simulink model "generator_loaded"  (R2021a)
settings: Solver=FixedStepAuto  StartTime=0.0  StopTime=5  FixedStep=1e-4  RelTol=1e-3
values from neighbouring files (symbols this model uses):
  f = 0.59e-4    (= 5.9e-05)    [generator_parameters.m]
  Ji = 1.15e-3    (= 0.00115)    [generator_parameters.m]
  ld = 5e-3    (= 0.005)    [generator_parameters.m]
  lq = 5e-3    (= 0.005)    [generator_parameters.m]
  p = 5    [generator_parameters.m]
  phi = 0.27    [generator_parameters.m]
  rs = 0.5    [generator_parameters.m]
libraries: spsControlledCurrentSourceLib x3, spsSeriesRLCBranchLib x3, spsVoltageMeasurementLib x3, spspowerguiLib x1
settings DebuggingCC: UnconnectedInputMsg=none  UnconnectedOutputMsg=none  UnconnectedLineMsg=none
settings ModelReferenceCC: EnableRefExpFcnMdlSchedulingChecks=off
settings RTWCC: Description=Generic Real-Time Target  DLArmComputeVersion=20.02.1

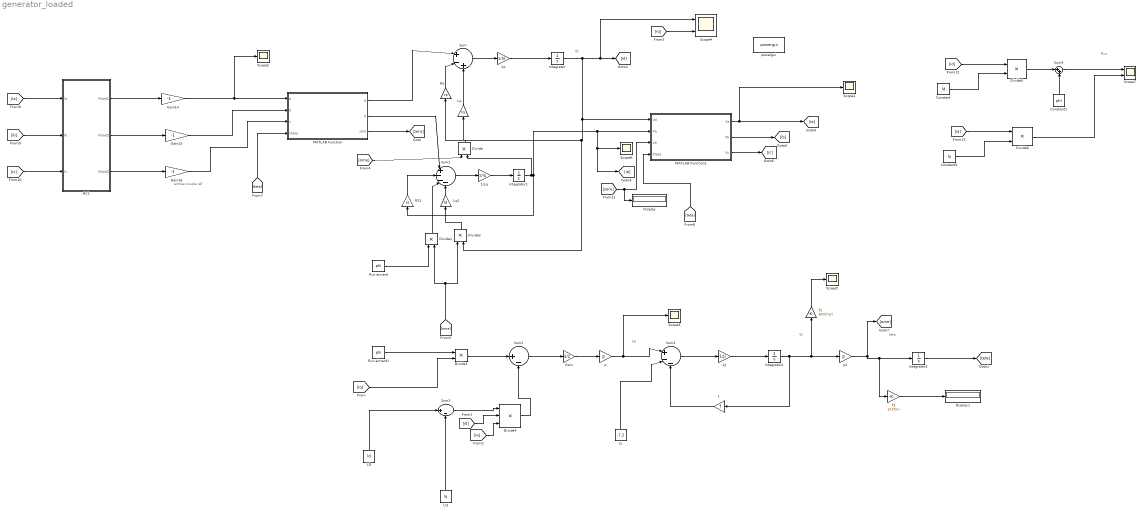
== system generator_loaded ==
  note: flux
  note: W
  note: ID
  note: entrée couple réf
  note: Ce
  note: teta
  1/L : Gain  Gain=1/ld
  1/Lq : Gain  Gain=1/lq
  1/j : Gain  Gain=1/Ji
  Constant : Constant  Value=ld
  Constant1 : Constant  Value=phi
  Constant2 : Constant  Value=lq
  Cr : Constant  Value=-7.2
  Display : Display
  Display1 : Display
  Divide{,1..3,5..6} (6 alike) : Product  Inputs=**
  Divide4 : Product  Inputs=***
  Gain : Gain  Gain=3/2
  Gain14 : Gain  Gain=-1
  Gain15 : Gain  Gain=-1
  Gain16 : Gain  Gain=-1
  Integrator : Integrator  InitialCondition=0.00001
  Integrator1 : Integrator
  Integrator2 : Integrator  InitialCondition=0.00001
  Integrator3 : Integrator
  LD : Constant  Value=ld
  LQ : Constant  Value=lq
  Lq : Gain  Gain=lq
  Lq1 : Gain  Gain=ld
  MATLAB Function : MATLAB Function  TreatAsAtomicUnit=on
  MATLAB Function1 : MATLAB Function  TreatAsAtomicUnit=on
  RC1 : Subsystem
  RS : Gain  Gain=rs
  RS1 : Gain  Gain=rs
  Scope{1..3,5..6} (5 alike) : Scope
  Scope4 : Scope  NumInputPorts=2
  Scope7 : Scope  NumInputPorts=2
  Sum : Sum  Inputs=|+-+
  Sum1 : Sum  Inputs=|+---
  Sum2 : Sum  Inputs=|+-
  Sum3 : Sum  Inputs=|+-
  Sum4 : Sum  Inputs=|+--
  Sum5 : Sum  Inputs=|++
  f : Gain  Gain=f
  f1 : Gain  Gain=60/(2*pi)
  f2 : Gain  Gain=1/(2*pi)
  flux aiment : Constant  Value=phi
  flux aiment1 : Constant  Value=phi
  p : Gain  Gain=p
  p1 : Gain  Gain=p
  powergui : spspowerguiLib/powergui  Priority=1  SimulationMode=Continuous  SampleTime=50e-6  frequency=60  Iterations=50  frequencyindice=0  Pbase=100e6  ErrMax=1e-4  UnitsV=kV  UnitsW=MW  buscounter=0  FunctionMessages=off  echomessages=off  EnableUseOfTLC=off  CurrentSourceSwitches=off  DisableSnubberDevices=off  DisableRonSwitches=off  DisableVfSwitches=off  DisplayEquations=off  AutomaticDiscreteSolvers=off  SolverType=Tustin/Backward Euler (TBE)  Interpol=off  ExternalGateDelay=off  methode=off  Ts=100  x0status=blocks  SPID=on  SwTol=0  HookPort=off  NonlinearTolerance=1e-4  nMaxIteration=100  ContinueOnMaxIteration=off  RestoreLinks=warning  ResistiveCurrentMeasurement=off  Frange=[0:2:500]  Ylog=off  Xlog=on  ShowGrid=off  save=off  variable=ZData  structure=0  ZoomFFT=off  StartTime=0.0  cycles=1  DisplayStyle=1  fundamental=60  FreqAxis=off  MaxFrequency=1000  frequencyindicesteady=1  RmsSteady=1  display=off
  wires:
  RC1/1(Vload1) -> Gain14/1
  RC1/2(Vload2) -> Gain15/1
  RC1/3(Vload3) -> Gain16/1
  Gain14/1 -> Scope2/1, MATLAB Function/1(a)
  Gain15/1 -> MATLAB Function/2(b)
  Gain16/1 -> MATLAB Function/3(c)
  MATLAB Function/1(d) -> Sum/1
  RS/1 -> Sum/2
  Lq/1 -> Sum/3
  Sum/1 -> 1/L/1
  Integrator/1 -> Scope4/1, [id], MATLAB Function1/1(Vd), Divide2/2, RS/1
  MATLAB Function/2(q) -> Sum1/1
  RS1/1 -> Sum1/2
  Sum1/1 -> 1/Lq/1
  Divide/1 -> Lq/1
  Integrator1/1 -> Divide/2, RS1/1, Scope6/1, [iq], MATLAB Function1/2(Vq)
  flux aiment/1 -> Divide1/1
  Divide1/1 -> Sum1/3
  Divide2/1 -> Lq1/1
  flux aiment1/1 -> Divide3/1
  Divide3/1 -> Sum2/1
  Sum3/1 -> Divide4/1
  [id] -> Divide4/2
  [iq] -> Divide4/3
  Divide4/1 -> Sum2/2
  Sum2/1 -> Gain/1
  Gain/1 -> p/1
  p/1 -> Scope3/1, Sum4/1
  Cr/1 -> Sum4/2
  Sum4/1 -> 1/j/1
  f/1 -> Sum4/3
  p1/1 -> f2/1, Integrator3/1, [ome]
  MATLAB Function1/1(Va) -> Scope1/1, [ia]
  MATLAB Function1/2(Vb) -> [ib]
  MATLAB Function1/3(Vc) -> [ic]
  [ia] -> RC1/1(Ia)
  [ib] -> RC1/2(Ib)
  [ic] -> RC1/3(Ic)
  MATLAB Function/3(zero) -> [zero]
  [zero] -> Display/1, MATLAB Function1/3(V0)
  1/Lq/1 -> Integrator1/1
  1/j/1 -> Integrator2/1
  1/L/1 -> Integrator/1
  [teta] -> MATLAB Function1/4(theta)
  [ome] -> Divide/1
  [ome] -> Divide2/1, Divide1/2
  [teta] -> MATLAB Function/4(theta)
  [iq] -> Divide3/2
  LD/1 -> Sum3/1
  LQ/1 -> Sum3/2
  Integrator3/1 -> [teta]
  Lq1/1 -> Sum1/4
  Integrator2/1 -> f1/1, p1/1, f/1
  f1/1 -> Scope5/1
  f2/1 -> Display1/1
  [iq] -> Scope4/2
  [id] -> Divide5/1
  Constant/1 -> Divide5/2
  Divide5/1 -> Sum5/1
  Constant1/1 -> Sum5/2
  [iq] -> Divide6/1
  Constant2/1 -> Divide6/2
  Divide6/1 -> Scope7/2
  Sum5/1 -> Scope7/1

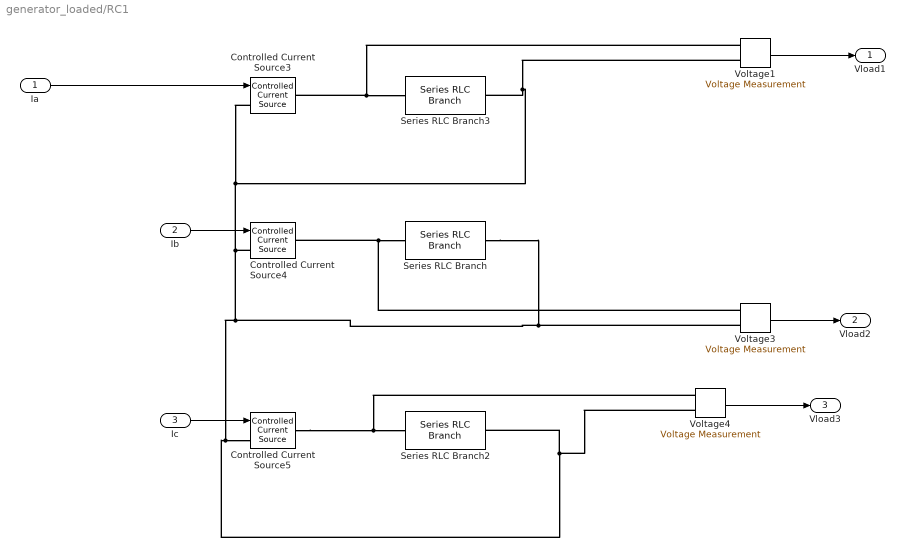
== system generator_loaded/RC1 ==
  Ia : Inport
  Ib : Inport  Port=2
  Ic : Inport  Port=3
  Controlled Current Source3 : spsControlledCurrentSourceLib/Controlled Current Source  Initialize=on  Source_Type=AC  Amplitude=0.1  Phase=0  Frequency=0  Measurements=Current
  Controlled Current Source4 : spsControlledCurrentSourceLib/Controlled Current Source  Initialize=on  Source_Type=AC  Amplitude=0.1  Phase=0  Frequency=0  Measurements=Current
  Controlled Current Source5 : spsControlledCurrentSourceLib/Controlled Current Source  Initialize=on  Source_Type=AC  Amplitude=0.1  Phase=0  Frequency=0  Measurements=Current
  Series RLC Branch : spsSeriesRLCBranchLib/Series RLC Branch  LConnTagsString=__new0  RConnTagsString=__new0  BranchType=R  Resistance=23  Inductance=1e-3  SetiL0=off  InitialCurrent=0  Capacitance=1e-6  Setx0=off  InitialVoltage=0  Measurements=None
  Series RLC Branch2 : spsSeriesRLCBranchLib/Series RLC Branch  LConnTagsString=__new0  RConnTagsString=__new0  BranchType=R  Resistance=23  Inductance=1e-3  SetiL0=off  InitialCurrent=0  Capacitance=1e-6  Setx0=off  InitialVoltage=0  Measurements=None
  Series RLC Branch3 : spsSeriesRLCBranchLib/Series RLC Branch  LConnTagsString=__new0  RConnTagsString=__new0  BranchType=R  Resistance=23  Inductance=1e-3  SetiL0=off  InitialCurrent=0  Capacitance=1e-6  Setx0=off  InitialVoltage=0  Measurements=None
  Voltage1 : spsVoltageMeasurementLib/Voltage Measurement  PhasorSimulation=off  OutputType=Complex  PSBequivalent=0
  Voltage3 : spsVoltageMeasurementLib/Voltage Measurement  PhasorSimulation=off  OutputType=Complex  PSBequivalent=0
  Voltage4 : spsVoltageMeasurementLib/Voltage Measurement  PhasorSimulation=off  OutputType=Complex  PSBequivalent=0
  Vload1 : Outport  VectorParamsAs1DForOutWhenUnconnected=off
  Vload2 : Outport  Port=2  VectorParamsAs1DForOutWhenUnconnected=off
  Vload3 : Outport  Port=3  VectorParamsAs1DForOutWhenUnconnected=off
  wires:
  Ib/1 -> Controlled Current Source4/1
  Ic/1 -> Controlled Current Source5/1
  Ia/1 -> Controlled Current Source3/1
  Voltage4/1 -> Vload3/1
  Voltage3/1 -> Vload2/1
  Voltage1/1 -> Vload1/1
  connections:
  Controlled Current Source3/RConn1 -- Voltage1/LConn1 -- Series RLC Branch3/LConn1
  Controlled Current Source5/RConn1 -- Voltage4/LConn1 -- Series RLC Branch2/LConn1
  Controlled Current Source4/LConn1 -- Series RLC Branch/RConn1 -- Voltage3/LConn2 -- Series RLC Branch2/RConn1 -- Voltage4/LConn2 -- Controlled Current Source5/LConn1 -- Controlled Current Source3/LConn1 -- Voltage1/LConn2 -- Series RLC Branch3/RConn1
  Voltage3/LConn1 -- Series RLC Branch/LConn1 -- Controlled Current Source4/RConn1

== matlab function generator_loaded/MATLAB Function1 ==
  data: Vd input; Va output; Vq input; V0 input; theta input; Vb output; Vc output
function [Va, Vb, Vc] = fcn(Vd, Vq, V0, theta)
    k = sqrt(2/3);
    homopolaire = V0 / sqrt(2); 
    Va = k * (Vd * cos(theta) - Vq * sin(theta) + homopolaire);
    Vb = k * (Vd * cos(theta - 2*pi/3) - Vq * sin(theta - 2*pi/3) + homopolaire);
    Vc = k * (Vd * cos(theta + 2*pi/3) - Vq * sin(theta + 2*pi/3) + homopolaire);
end

== matlab function generator_loaded/MATLAB Function ==
  data: a input; d output; b input; c input; theta input; q output; zero output
function [d, q, zero] = fcn(a, b, c, theta)

    d = sqrt(2/3) * (a*cos(theta) + b*cos(theta - 2*pi/3) + c*cos(theta + 2*pi/3));
    q = sqrt(2/3) * (-a*sin(theta) - b*sin(theta - 2*pi/3) - c*sin(theta + 2*pi/3));
    zero = sqrt(1/3) * (a + b + c);
end
